simulink model "GA_PowerSystems"  (R2024a)
settings: Solver=VariableStepAuto  StartTime=0.0  StopTime=0.5  RelTol=1e-3
undefined symbols (not defined in the file or in its folder): D1, Delta
libraries: spsRMSLib x3, simulink_extras x3, spsThreePhaseVIMeasurementLib x2, spsDistributedParametersLineLib x1, spsThreePhaseParallelRLCLoadLib x1, spsThreePhaseTransformerTwoWindingsLib x1, spsThreePhaseBreakerLib x1, spsThreePhaseFaultLib x1, spsThreePhaseSourceLib x1, sps_lib x1
settings Model: Creator=nnete  LastModifiedBy=nnete

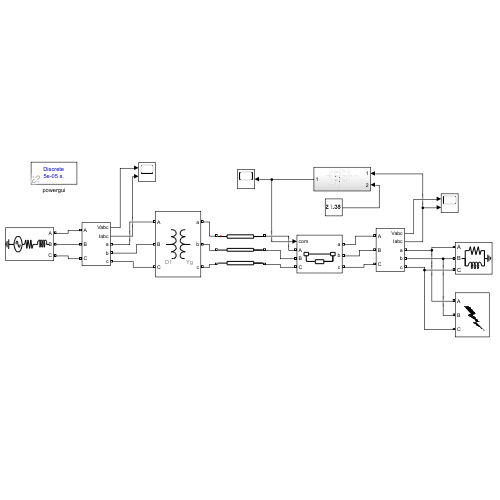
[thumbnail: Simulink's stored preview of the top-level diagram]
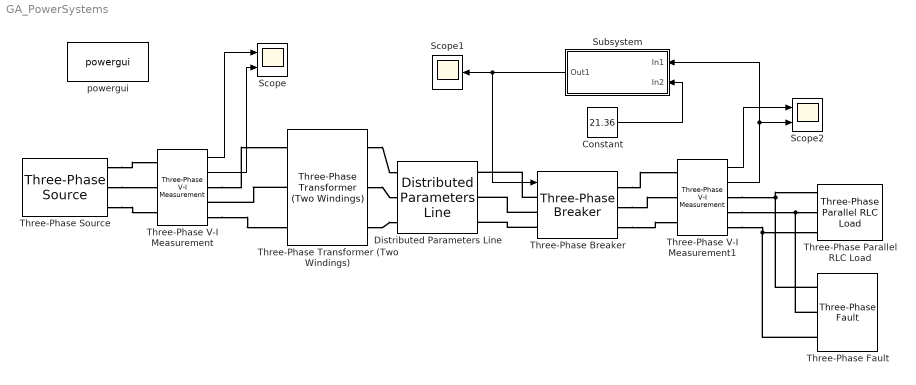
== system GA_PowerSystems ==
  Constant : Constant  Value=21.36
  Distributed Parameters Line : spsDistributedParametersLineLib/Distributed Parameters Line  Phases=3  Length=47.8  Frequency=50  Resistance=[0.01273 0.3864]  Inductance="[0.9337e-3  4.1264e-3]"  Capacitance=[12.74e-9 7.751e-9]  x1=[-0.0003 -7.57778156341323e-12 337.330116249299 -240.250086830447;-0.00025 -7.66965291458836e-12 341.062185018035 -234.921896598693;-0.0002 -7.75963189367029e-12 344.71010179604 -229.535742904166;-0.00015 -7.84769629969233e-12 348.272966514435 -224.092954699694;-0.0001 -7.93382440408002e-12 351.749900089663 -218.594874911824;-5e-05 -8.01799495601236e-12 355.140044640391 -213.042860109475]  x2=[-0.0003 1.62502004253353e-10 -1.008916717381 -43.23374080033;-0.00025 1.69531356353004e-10 -0.329706164508055 -43.2442545360579;-0.0002 1.76518879127227e-10 0.349585738427481 -43.2440983990568;-0.00015 1.83462848509334e-10 1.02879138631302 -43.233272427851;-0.0001 1.90361551178785e-10 1.70774319531813 -43.2117792935869;-5e-05 1.97213284983924e-10 2.3862736442433 -43.179624299374]  x3=[-0.0003 -5.92665697231726e-12 14.1924648493174 23.7586164228428;-0.00025 -5.85568953845455e-12 13.8175298331076 23.9786109301201;-0.0002 -5.78327730081879e-12 13.4391855481677 24.1926890739501;-0.00015 -5.7094381260461e-12 13.0575253452886 24.4007980337541;-0.0001 -5.63419023284795e-12 12.6726433934144 24.6028864617601;-5e-05 -5.55755218751605e-12 12.2846346564078 24.7989044956727]  x4=[-0.0003 6.11607928475798e-12 -12.9793253196863 -24.8361460094091;-0.00025 6.05459890721107e-12 -12.5876148663606 -25.036952417;-0.0002 5.99162464798071e-12 -12.1927986074192 -25.231581331218;-0.00015 5.92717204502307e-12 -11.7949739578662 -25.4199847302908;-0.0001 5.8612570010535e-12 -11.394239074981 -25.6021161284988;-5e-05 5.79389577962278e-12 -10.9906928340998 -25.7779305876447]  x5=0.000270328869023965  V1=ones(3,3)  V2=ones(3,3)  I1=ones(3,3)  I2=ones(3,3)  nHarmo=1  Measurements=None  Decoupling=off  VsMag0=0  VrMag0=0  VsAngle0=0  VrAngle0=0  IsMag0=0  IrMag0=0  IsAngle0=0  IrAngle0=0
      settings: LibrarySourceBlock=sps_lib/Power Grid Elements/Distributed Parameters Line
  Scope : Scope  NumInputPorts=2
  Scope1 : Scope
  Scope2 : Scope  NumInputPorts=2
  Subsystem : Subsystem
  Three-Phase Parallel RLC Load : spsThreePhaseParallelRLCLoadLib/Three-Phase Parallel RLC Load  LConnTagsString=A|B|C  Configuration=Y (grounded)  NominalVoltage=415  Vabc=[1e3 1e3 1e3]  Vabcp=[1e3 1e3 1e3]  NominalFrequency=50  UnbalancedPower=off  ActivePower=100e3  InductivePower=50e3  CapacitivePower=0  Pabc=[10e3 9e3 11e3]  QLabc=[100 90 110]  QCabc=[100 90 110]  Pabcp=[10e3 9e3 11e3]  QLabcp=[100 90 110]  QCabcp=[100 90 110]  Measurements=None  LoadType=constant Z
  Three-Phase Transformer (Two Windings) : spsThreePhaseTransformerTwoWindingsLib/Three-Phase Transformer (Two Windings)  Winding1Connection=Delta (D1)  Winding2Connection=Yg  CoreType=Three single-phase transformers  SetSaturation=off  Hysteresis=off  DataFile='hysteresis'  SetInitialFlux=off  Measurements=None  UNITS=pu  NominalPower=[ 10e6 , 50 ]  Winding1=[ 11e3 , 0.002 , 0.08 ]  Winding2=[ 415 , 0.002 , 0.08 ]  Rm=500  Lm=500  L0=0.5  Saturation=[ 0,0 ; 0.0024,1.2 ; 1.0,1.52 ]  InitialFluxes=[0.8 -0.8 0.7]  BreakLoop=off  DiscreteSolver=Trapezoidal iterative  DataType=off  TransfoNumber=1
  Three-Phase V-I Measurement : spsThreePhaseVIMeasurementLib/Three-Phase V-I Measurement  VoltageMeasurement=phase-to-phase  SetLabelV=off  LabelV=Vabc  Vpu=off  VpuLL=off  CurrentMeasurement=yes  SetLabelI=off  LabelI=Iabc  Ipu=off  Pbase=100e6  Vbase=500e3  OutputType=Complex  PhasorSimulation=off  PSBequivalent=0
  Three-Phase V-I Measurement1 : spsThreePhaseVIMeasurementLib/Three-Phase V-I Measurement  VoltageMeasurement=phase-to-phase  SetLabelV=off  LabelV=Vabc  Vpu=off  VpuLL=off  CurrentMeasurement=yes  SetLabelI=off  LabelI=Iabc  Ipu=off  Pbase=100e6  Vbase=500e3  OutputType=Complex  PhasorSimulation=off  PSBequivalent=0
  Three-Phase Breaker : spsThreePhaseBreakerLib/Three-Phase Breaker  InitialState=closed  SwitchA=on  SwitchB=on  SwitchC=on  SwitchTimes="[1/60  5/60]"  External=on  BreakerResistance=0.01  SnubberResistance=1e6  SnubberCapacitance=inf  Measurements=None
  Three-Phase Fault : spsThreePhaseFaultLib/Three-Phase Fault  InitialStates=0  FaultA=on  FaultB=on  FaultC=on  GroundFault=off  SwitchTimes="[5/50  10/50]"  External=off  SwitchStatus=NaN  FaultResistance=0.001  GroundResistance=0.01  SnubberResistance=1e6  SnubberCapacitance=inf  Measurements=Fault currents
  Three-Phase Source : spsThreePhaseSourceLib/Three-Phase Source  InternalConnection=Yg  VoltagePhases=off  Voltage=11e3  PhaseAngle=0  Voltage_phases=[25e3 25e3 25e3]/sqrt(3)  PhaseAngles_phases=[0 -120 +120]  Frequency=50  NonIdealSource=on  SpecifyImpedance=on  Resistance=0.8929  Inductance=16.58e-3  ShortCircuitLevel=20e6  BaseVoltage=11e3  XRratio=7  BusType=swing  Pref=10e3  Qref=0  Prefabc=[10e3, 10e3, 10e3]  Qrefabc=[0, 0, 0]  Qmin=-inf  Qmax=inf
  powergui : sps_lib/powergui  Priority=1  SimulationMode=Discrete  SampleTime=50e-06  frequency=60  Iterations=50  frequencyindice=50  Pbase=100e6  ErrMax=1e-4  UnitsV=kV  UnitsW=MW  buscounter=0  FunctionMessages=off  echomessages=off  EnableUseOfTLC=off  CurrentSourceSwitches=off  DisableSnubberDevices=off  DisableRonSwitches=off  DisableVfSwitches=off  DisplayEquations=off  AutomaticDiscreteSolvers=off  SolverType=Tustin/Backward Euler (TBE)  Interpol=off  ExternalGateDelay=off  methode=off  Ts=100  x0status=blocks  SPID=on  SwTol=0  HookPort=off  NonlinearTolerance=1e-4  nMaxIteration=100  ContinueOnMaxIteration=off  RestoreLinks=warning  ResistiveCurrentMeasurement=off  Frange=[0:2:500]  Ylog=off  Xlog=on  ShowGrid=off  save=off  variable=ZData  structure=0  ZoomFFT=off  StartTime=0.0  cycles=1  DisplayStyle=1  fundamental=60  FreqAxis=off  MaxFrequency=1000  frequencyindicesteady=1  RmsSteady=1  display=off
  wires:
  Subsystem/1(Out1) -> Scope1/1, Three-Phase Breaker/1
  Constant/1 -> Subsystem/2(In2)
  Three-Phase V-I Measurement/1 -> Scope/1
  Three-Phase V-I Measurement/2 -> Scope/2
  Three-Phase V-I Measurement1/1 -> Scope2/1
  Three-Phase V-I Measurement1/2 -> Subsystem/1(In1), Scope2/2
  connections:
  Three-Phase Source/RConn1 -- Three-Phase V-I Measurement/LConn1
  Three-Phase Source/RConn2 -- Three-Phase V-I Measurement/LConn2
  Three-Phase Source/RConn3 -- Three-Phase V-I Measurement/LConn3
  Three-Phase Transformer (Two Windings)/LConn2 -- Three-Phase V-I Measurement/RConn2
  Three-Phase V-I Measurement/RConn3 -- Three-Phase Transformer (Two Windings)/LConn3
  Three-Phase V-I Measurement/RConn1 -- Three-Phase Transformer (Two Windings)/LConn1
  Three-Phase Transformer (Two Windings)/RConn2 -- Distributed Parameters Line/LConn2
  Three-Phase Transformer (Two Windings)/RConn3 -- Distributed Parameters Line/LConn3
  Three-Phase Transformer (Two Windings)/RConn1 -- Distributed Parameters Line/LConn1
  Three-Phase Breaker/LConn1 -- Distributed Parameters Line/RConn1
  Three-Phase Breaker/LConn2 -- Distributed Parameters Line/RConn2
  Three-Phase Breaker/LConn3 -- Distributed Parameters Line/RConn3
  Three-Phase V-I Measurement1/RConn1 -- Three-Phase Parallel RLC Load/LConn1 -- Three-Phase Fault/LConn1
  Three-Phase V-I Measurement1/RConn2 -- Three-Phase Fault/LConn2 -- Three-Phase Parallel RLC Load/LConn2
  Three-Phase V-I Measurement1/RConn3 -- Three-Phase Fault/LConn3 -- Three-Phase Parallel RLC Load/LConn3
  Three-Phase Breaker/RConn1 -- Three-Phase V-I Measurement1/LConn1
  Three-Phase Breaker/RConn2 -- Three-Phase V-I Measurement1/LConn2
  Three-Phase Breaker/RConn3 -- Three-Phase V-I Measurement1/LConn3

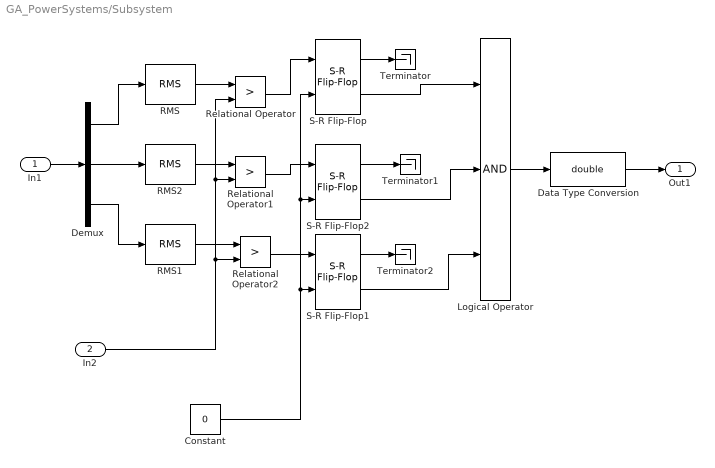
== system GA_PowerSystems/Subsystem ==
  In1 : Inport
  In2 : Inport  Port=2
  Constant : Constant  Value=0  OutDataTypeStr=boolean
  Data Type Conversion : DataTypeConversion  OutDataTypeStr=double  SaturateOnIntegerOverflow=off  RndMeth=Floor
  Demux : Demux  Outputs=3
  Logical Operator : Logic  Inputs=3  AllPortsSameDT=off  OutDataTypeStr=boolean
  RMS : spsRMSLib/RMS  TrueRMS=on  Freq=50  RMSInit=0  Ts=0.01
  RMS1 : spsRMSLib/RMS  TrueRMS=on  Freq=50  RMSInit=0  Ts=0.01
  RMS2 : spsRMSLib/RMS  TrueRMS=on  Freq=50  RMSInit=0  Ts=0.01
  Relational Operator : RelationalOperator  Operator=>  OutDataTypeStr=boolean  RndMeth=Simplest  InputSameDT=off
  Relational Operator1 : RelationalOperator  Operator=>  OutDataTypeStr=boolean  RndMeth=Simplest  InputSameDT=off
  Relational Operator2 : RelationalOperator  Operator=>  OutDataTypeStr=boolean  RndMeth=Simplest  InputSameDT=off
  S-R Flip-Flop : simulink_extras/Flip Flops/S-R Flip-Flop  initial_condition=0
  S-R Flip-Flop1 : simulink_extras/Flip Flops/S-R Flip-Flop  initial_condition=0
  S-R Flip-Flop2 : simulink_extras/Flip Flops/S-R Flip-Flop  initial_condition=0
  Terminator : Terminator
  Terminator1 : Terminator
  Terminator2 : Terminator
  Out1 : Outport
  wires:
  In1/1 -> Demux/1
  Demux/2 -> RMS2/1
  Demux/3 -> RMS1/1
  Demux/1 -> RMS/1
  RMS/1 -> Relational Operator/1
  RMS2/1 -> Relational Operator1/1
  Relational Operator/1 -> S-R Flip-Flop/1
  Relational Operator1/1 -> S-R Flip-Flop2/1
  Relational Operator2/1 -> S-R Flip-Flop1/1
  Logical Operator/1 -> Data Type Conversion/1
  Data Type Conversion/1 -> Out1/1
  S-R Flip-Flop/1 -> Terminator/1
  S-R Flip-Flop2/1 -> Terminator1/1
  S-R Flip-Flop1/1 -> Terminator2/1
  S-R Flip-Flop1/2 -> Logical Operator/3
  S-R Flip-Flop2/2 -> Logical Operator/2
  S-R Flip-Flop/2 -> Logical Operator/1
  RMS1/1 -> Relational Operator2/1
  In2/1 -> Relational Operator2/2, Relational Operator1/2, Relational Operator/2
  Constant/1 -> S-R Flip-Flop2/2, S-R Flip-Flop/2, S-R Flip-Flop1/2
